simulink model "ModelInterleavedBoostPFCController"  (R2026a)
settings: Solver=ode23t  StopTime=0.02  MaxStep=1e-5  AbsTol=1e-3
PreLoadFcn:
  | InterleavedBoostPFCDefaultInputParameters;
model workspace (MAT data in the model file):
  ConverterKey : string (value not decoded)
undefined symbols (not defined in the file or in its folder): interleavedController, interleavedDesign, Vref
libraries: fl_lib x32, ee_lib x21, nesl_utility x19, ConverterLibrary x1
(part 3 of 3)

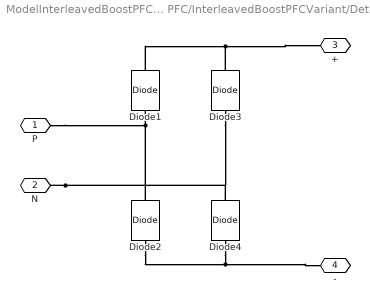
== system ModelInterleavedBoostPFCController/Interleaved Boost PFC/InterleavedBoostPFCVariant/DetailedModel/RectifierBridge/TabulatedDiode ==
  Diode1 : ee_lib/Semiconductors & Converters/Diode  PartSpecification="{\"CollectionId\":\"SimscapeElectrical\",\"CollectionVersion\":\"1.0.0\",\"DatasetId\":\"Infineon|IDW80C65D1|simscape.electrical.diode\",\"DisplayName\":\"Infineon:IDW80C65D1\"}"  ModelType=ee.enum.diode.modelType.tabulated  TableType=ee.enum.diode.tableType.IfMat  IfMat=[0.0001 0.0001 0.1601 0.6065 1.9426 5.4603 12.2546 21.9425 34.4556 49.1982 64.7538 83.3404;0.3114 0.8503 2.3479 5.2232 9.8335 15.9488 23.5801 32.5233 43.1998 54.3228 66.653 79.8979] % Datasheet derived A  VfMat=[.9, 1.15, 1.25, 1.5, 1.75, 2.17, 2.6, 2.85; .58, .68, .75, 1.1, 1.38, 1.77, 2.27, 2.7] % Parameter not set V  TjVec=[25 175] % Datasheet derived degC  VfVec=[0.3258 0.4465 0.5672 0.6878 0.8085 0.9292 1.0498 1.1705 1.2912 1.4118 1.5325 1.6532] % Datasheet derived V  IfVec=[.1, .2, .5, 1, 2, 4, 7, 10] % Parameter not set A  IrMat=[1e-06, 2e-06, 5e-06, 1e-05, 2.5e-05, 5e-05, .0001; 2e-06, 5e-06, 1e-05, 4e-05, 8e-05, .0002, .0005] % Parameter not set A  VrMat=[10, 100, 200, 250, 300, 325, 350; 10, 70, 160, 220, 270, 300, 320] % Parameter not set V  VrVec=[10, 20, 40, 50, 70, 80, 100] % Parameter not set V  IrVec=[1e-06, 2e-06, 5e-06, 1e-05, 2e-05, 5e-05, .0001] % Parameter not set A  Vf=0.6 % Parameter not set V  Ron=0.3 % Parameter not set Ohm  Goff=1e-08 % Parameter not set S  prmExp=ee.enum.diode.expParam.useTwo  I12=[.0137, .545] % Parameter not set A  V12=[.6, .7] % Parameter not set V  RS=0 % Parameter not set Ohm  Tmeas=298.15 % Parameter not set K  IS=1e-12 % Parameter not set A  ec=1 % Parameter not set  I1=0.0137 % Parameter not set A  V1=0.6 % Parameter not set V  N_series=1 % Parameter not set  N_parallel=1 % Parameter not set  ZenerEnable=false % Parameter not set  Rz=0.3 % Parameter not set Ohm  BV=inf % Parameter not set V  C_param=ee.enum.diode.capParam.fixed  CJ=5 pF  CJ0=5 % Parameter not set pF  Vvec=[.1, 10, 100] % Parameter not set V  Cvec=[3.5, 1, .4] % Parameter not set pF  VJ=1 % Parameter not set V  Mgrad=0.5 % Parameter not set  FC=0.5 % Parameter not set  Q_param=ee.enum.diode.recoveryParam.off  iRM=-7.15 % Parameter not set A  iF=4 % Parameter not set A  didt=-750 % Parameter not set A/us  trr_factor=3 % Parameter not set  trr=115 % Parameter not set ns  Qrr=150 % Parameter not set nA*s  Vr=-600 % Parameter not set V  Ls=150 % Parameter not set nH  Erec=0.03 % Parameter not set J  TT=50 % Parameter not set ns  tau=100 % Parameter not set ns  T_param=ee.enum.diode.temperatureParam.off  Tdevice=simTemp_K K  I1_T2=0.245 % Parameter not set A  V1_T2=0.5 % Parameter not set V  IS_T2=1.25e-7 % Parameter not set A  Tmeas2=125 % Parameter not set degC  XTI_param=ee.enum.diode.xtiParam.pn  XTI=3 % Parameter not set  EG_param=ee.enum.diode.egapParam.material_si  EG=1.11 % Parameter not set eV  dBVdT=0 % Parameter not set V/K  enable_fault_input=simscape.enum.onoff.off  i_specify=off  i_priority=None  i=0 A  i_nominal_specify=off  i_nominal_value=1  i_nominal_unit=A  v_specify=off  v_priority=None  v=0 V  v_nominal_specify=off  v_nominal_value=1  v_nominal_unit=V  v_capacitor_specify=off  v_capacitor_priority=None  v_capacitor=0 V  v_capacitor_nominal_specify=off  v_capacitor_nominal_value=1  v_capacitor_nominal_unit=V  Qj_specify=off  Qj_priority=High  Qj=0 C  Qj_nominal_specify=off  Qj_nominal_value=1  Qj_nominal_unit=C  i_diode_specify=off  i_diode_priority=None  i_diode=0 A  i_diode_nominal_specify=off  i_diode_nominal_value=1  i_diode_nominal_unit=A  v_diode_specify=off  v_diode_priority=None  v_diode=0 V  v_diode_nominal_specify=off  v_diode_nominal_value=1  v_diode_nominal_unit=V  i_capacitor_specify=off  i_capacitor_priority=None  i_capacitor=0 A  i_capacitor_nominal_specify=off  i_capacitor_nominal_value=1  i_capacitor_nominal_unit=A  fidelity_level=ee.enum.diode.fidelity.includeChargeDyn  rec_loss_model=ee.enum.diode.reverseRecoveryModel.fixed  ErecVal=0 % Parameter not set J  scaleWithIandV=true % Parameter not set  ErecMat=zeros(2, 3) % Parameter not set J  ErecMat3D=zeros(2, 3, 2) J  TjrecVec=[298.15, 398.15] % Parameter not set K  IfrecVec=[.1, 1, 10] % Parameter not set A  IrecVal=10 % Parameter not set A  VrecVal=10 % Parameter not set V  VrecVec=[0, 100] V  tFilter=1 / 1000 / 100 % Parameter not set s  thermal_network_parameterization=ee.enum.thermalNetworkTopology.junctionCase  Rth=[0, 10] % Parameter not set K/W  Rth_Cauer=[1, 3, 10] % Parameter not set K/W  Rth_Foster=[.08, .14, .22, .16] % Parameter not set K/W  thermal_mass_parameterization=ee.enum.thermalNetwork.timeconstant  thermal_mass=[0, 1] % Parameter not set J/K  thermal_mass_Cauer=[.1, .3, 1] % Parameter not set J/K  thermal_mass_Foster=[.001, .005, .05, .5] % Parameter not set J/K  thermal_time_constant=[0, 10] % Parameter not set s  thermal_time_constant_Cauer=[1, 3, 10] % Parameter not set s  thermal_time_constant_Foster=[7e-05, .0007, .01, .08] % Parameter not set s  thermal_mass_initial_temperatures=[25, 25] % Parameter not set degC  thermal_mass_initial_temperatures_Cauer=[25, 25, 25] % Parameter not set degC  junction_thermal_mass=0.01 % Parameter not set J/K  Tvec_initial_Foster=[25, 25, 25, 25] % Parameter not set degC  no_thermal_network=0 % Parameter not set  junction_temperature_specify=off  junction_temperature_priority=None  junction_temperature=25 degC  junction_temperature_nominal_specify=off  junction_temperature_nominal_value=1  junction_temperature_nominal_unit=degC
      settings: AttributesFormatString=Infineon:IDW80C65D1
  Diode2 : ee_lib/Semiconductors & Converters/Diode  ModelType=ee.enum.diode.modelType.tabulated  TableType=ee.enum.diode.tableType.IfMat  IfMat=[0.0001 0.0001 0.1601 0.6065 1.9426 5.4603 12.2546 21.9425 34.4556 49.1982 64.7538 83.3404;0.3114 0.8503 2.3479 5.2232 9.8335 15.9488 23.5801 32.5233 43.1998 54.3228 66.653 79.8979] % Datasheet derived A  VfMat=[.9, 1.15, 1.25, 1.5, 1.75, 2.17, 2.6, 2.85; .58, .68, .75, 1.1, 1.38, 1.77, 2.27, 2.7] % Parameter not set V  TjVec=[25 175] % Datasheet derived degC  VfVec=[0.3258 0.4465 0.5672 0.6878 0.8085 0.9292 1.0498 1.1705 1.2912 1.4118 1.5325 1.6532] % Datasheet derived V  IfVec=[.1, .2, .5, 1, 2, 4, 7, 10] % Parameter not set A  IrMat=[1e-06, 2e-06, 5e-06, 1e-05, 2.5e-05, 5e-05, .0001; 2e-06, 5e-06, 1e-05, 4e-05, 8e-05, .0002, .0005] % Parameter not set A  VrMat=[10, 100, 200, 250, 300, 325, 350; 10, 70, 160, 220, 270, 300, 320] % Parameter not set V  VrVec=[10, 20, 40, 50, 70, 80, 100] % Parameter not set V  IrVec=[1e-06, 2e-06, 5e-06, 1e-05, 2e-05, 5e-05, .0001] % Parameter not set A  Vf=0.6 % Parameter not set V  Ron=0.3 % Parameter not set Ohm  Goff=1e-08 % Parameter not set S  prmExp=ee.enum.diode.expParam.useTwo  I12=[.0137, .545] % Parameter not set A  V12=[.6, .7] % Parameter not set V  RS=0 % Parameter not set Ohm  Tmeas=298.15 % Parameter not set K  IS=1e-12 % Parameter not set A  ec=1 % Parameter not set  I1=0.0137 % Parameter not set A  V1=0.6 % Parameter not set V  N_series=1 % Parameter not set  N_parallel=1 % Parameter not set  ZenerEnable=false % Parameter not set  Rz=0.3 % Parameter not set Ohm  BV=inf % Parameter not set V  C_param=ee.enum.diode.capParam.fixed  CJ=5 pF  CJ0=5 % Parameter not set pF  Vvec=[.1, 10, 100] % Parameter not set V  Cvec=[3.5, 1, .4] % Parameter not set pF  VJ=1 % Parameter not set V  Mgrad=0.5 % Parameter not set  FC=0.5 % Parameter not set  Q_param=ee.enum.diode.recoveryParam.off  iRM=-7.15 % Parameter not set A  iF=4 % Parameter not set A  didt=-750 % Parameter not set A/us  trr_factor=3 % Parameter not set  trr=115 % Parameter not set ns  Qrr=150 % Parameter not set nA*s  Vr=-600 % Parameter not set V  Ls=150 % Parameter not set nH  Erec=0.03 % Parameter not set J  TT=50 % Parameter not set ns  tau=100 % Parameter not set ns  T_param=ee.enum.diode.temperatureParam.off  Tdevice=simTemp_K K  I1_T2=0.245 % Parameter not set A  V1_T2=0.5 % Parameter not set V  IS_T2=1.25e-7 % Parameter not set A  Tmeas2=125 % Parameter not set degC  XTI_param=ee.enum.diode.xtiParam.pn  XTI=3 % Parameter not set  EG_param=ee.enum.diode.egapParam.material_si  EG=1.11 % Parameter not set eV  dBVdT=0 % Parameter not set V/K  enable_fault_input=simscape.enum.onoff.off  i_specify=off  i_priority=None  i=0 A  i_nominal_specify=off  i_nominal_value=1  i_nominal_unit=A  v_specify=off  v_priority=None  v=0 V  v_nominal_specify=off  v_nominal_value=1  v_nominal_unit=V  v_capacitor_specify=off  v_capacitor_priority=None  v_capacitor=0 V  v_capacitor_nominal_specify=off  v_capacitor_nominal_value=1  v_capacitor_nominal_unit=V  Qj_specify=off  Qj_priority=High  Qj=0 C  Qj_nominal_specify=off  Qj_nominal_value=1  Qj_nominal_unit=C  i_diode_specify=off  i_diode_priority=None  i_diode=0 A  i_diode_nominal_specify=off  i_diode_nominal_value=1  i_diode_nominal_unit=A  v_diode_specify=off  v_diode_priority=None  v_diode=0 V  v_diode_nominal_specify=off  v_diode_nominal_value=1  v_diode_nominal_unit=V  i_capacitor_specify=off  i_capacitor_priority=None  i_capacitor=0 A  i_capacitor_nominal_specify=off  i_capacitor_nominal_value=1  i_capacitor_nominal_unit=A  fidelity_level=ee.enum.diode.fidelity.includeChargeDyn  rec_loss_model=ee.enum.diode.reverseRecoveryModel.fixed  ErecVal=0 % Parameter not set J  scaleWithIandV=true % Parameter not set  ErecMat=zeros(2, 3) % Parameter not set J  ErecMat3D=zeros(2, 3, 2) J  TjrecVec=[298.15, 398.15] % Parameter not set K  IfrecVec=[.1, 1, 10] % Parameter not set A  IrecVal=10 % Parameter not set A  VrecVal=10 % Parameter not set V  VrecVec=[0, 100] V  tFilter=1 / 1000 / 100 % Parameter not set s  thermal_network_parameterization=ee.enum.thermalNetworkTopology.junctionCase  Rth=[0, 10] % Parameter not set K/W  Rth_Cauer=[1, 3, 10] % Parameter not set K/W  Rth_Foster=[.08, .14, .22, .16] % Parameter not set K/W  thermal_mass_parameterization=ee.enum.thermalNetwork.timeconstant  thermal_mass=[0, 1] % Parameter not set J/K  thermal_mass_Cauer=[.1, .3, 1] % Parameter not set J/K  thermal_mass_Foster=[.001, .005, .05, .5] % Parameter not set J/K  thermal_time_constant=[0, 10] % Parameter not set s  thermal_time_constant_Cauer=[1, 3, 10] % Parameter not set s  thermal_time_constant_Foster=[7e-05, .0007, .01, .08] % Parameter not set s  thermal_mass_initial_temperatures=[25, 25] % Parameter not set degC  thermal_mass_initial_temperatures_Cauer=[25, 25, 25] % Parameter not set degC  junction_thermal_mass=0.01 % Parameter not set J/K  Tvec_initial_Foster=[25, 25, 25, 25] % Parameter not set degC  no_thermal_network=0 % Parameter not set  junction_temperature_specify=off  junction_temperature_priority=None  junction_temperature=25 degC  junction_temperature_nominal_specify=off  junction_temperature_nominal_value=1  junction_temperature_nominal_unit=degC
  Diode3 : ee_lib/Semiconductors & Converters/Diode  ModelType=ee.enum.diode.modelType.tabulated  TableType=ee.enum.diode.tableType.IfMat  IfMat=[0.0001 0.0001 0.1601 0.6065 1.9426 5.4603 12.2546 21.9425 34.4556 49.1982 64.7538 83.3404;0.3114 0.8503 2.3479 5.2232 9.8335 15.9488 23.5801 32.5233 43.1998 54.3228 66.653 79.8979] % Datasheet derived A  VfMat=[.9, 1.15, 1.25, 1.5, 1.75, 2.17, 2.6, 2.85; .58, .68, .75, 1.1, 1.38, 1.77, 2.27, 2.7] % Parameter not set V  TjVec=[25 175] % Datasheet derived degC  VfVec=[0.3258 0.4465 0.5672 0.6878 0.8085 0.9292 1.0498 1.1705 1.2912 1.4118 1.5325 1.6532] % Datasheet derived V  IfVec=[.1, .2, .5, 1, 2, 4, 7, 10] % Parameter not set A  IrMat=[1e-06, 2e-06, 5e-06, 1e-05, 2.5e-05, 5e-05, .0001; 2e-06, 5e-06, 1e-05, 4e-05, 8e-05, .0002, .0005] % Parameter not set A  VrMat=[10, 100, 200, 250, 300, 325, 350; 10, 70, 160, 220, 270, 300, 320] % Parameter not set V  VrVec=[10, 20, 40, 50, 70, 80, 100] % Parameter not set V  IrVec=[1e-06, 2e-06, 5e-06, 1e-05, 2e-05, 5e-05, .0001] % Parameter not set A  Vf=0.6 % Parameter not set V  Ron=0.3 % Parameter not set Ohm  Goff=1e-08 % Parameter not set S  prmExp=ee.enum.diode.expParam.useTwo  I12=[.0137, .545] % Parameter not set A  V12=[.6, .7] % Parameter not set V  RS=0 % Parameter not set Ohm  Tmeas=298.15 % Parameter not set K  IS=1e-12 % Parameter not set A  ec=1 % Parameter not set  I1=0.0137 % Parameter not set A  V1=0.6 % Parameter not set V  N_series=1 % Parameter not set  N_parallel=1 % Parameter not set  ZenerEnable=false % Parameter not set  Rz=0.3 % Parameter not set Ohm  BV=inf % Parameter not set V  C_param=ee.enum.diode.capParam.fixed  CJ=5 pF  CJ0=5 % Parameter not set pF  Vvec=[.1, 10, 100] % Parameter not set V  Cvec=[3.5, 1, .4] % Parameter not set pF  VJ=1 % Parameter not set V  Mgrad=0.5 % Parameter not set  FC=0.5 % Parameter not set  Q_param=ee.enum.diode.recoveryParam.off  iRM=-7.15 % Parameter not set A  iF=4 % Parameter not set A  didt=-750 % Parameter not set A/us  trr_factor=3 % Parameter not set  trr=115 % Parameter not set ns  Qrr=150 % Parameter not set nA*s  Vr=-600 % Parameter not set V  Ls=150 % Parameter not set nH  Erec=0.03 % Parameter not set J  TT=50 % Parameter not set ns  tau=100 % Parameter not set ns  T_param=ee.enum.diode.temperatureParam.off  Tdevice=simTemp_K K  I1_T2=0.245 % Parameter not set A  V1_T2=0.5 % Parameter not set V  IS_T2=1.25e-7 % Parameter not set A  Tmeas2=125 % Parameter not set degC  XTI_param=ee.enum.diode.xtiParam.pn  XTI=3 % Parameter not set  EG_param=ee.enum.diode.egapParam.material_si  EG=1.11 % Parameter not set eV  dBVdT=0 % Parameter not set V/K  enable_fault_input=simscape.enum.onoff.off  i_specify=off  i_priority=None  i=0 A  i_nominal_specify=off  i_nominal_value=1  i_nominal_unit=A  v_specify=off  v_priority=None  v=0 V  v_nominal_specify=off  v_nominal_value=1  v_nominal_unit=V  v_capacitor_specify=off  v_capacitor_priority=None  v_capacitor=0 V  v_capacitor_nominal_specify=off  v_capacitor_nominal_value=1  v_capacitor_nominal_unit=V  Qj_specify=off  Qj_priority=High  Qj=0 C  Qj_nominal_specify=off  Qj_nominal_value=1  Qj_nominal_unit=C  i_diode_specify=off  i_diode_priority=None  i_diode=0 A  i_diode_nominal_specify=off  i_diode_nominal_value=1  i_diode_nominal_unit=A  v_diode_specify=off  v_diode_priority=None  v_diode=0 V  v_diode_nominal_specify=off  v_diode_nominal_value=1  v_diode_nominal_unit=V  i_capacitor_specify=off  i_capacitor_priority=None  i_capacitor=0 A  i_capacitor_nominal_specify=off  i_capacitor_nominal_value=1  i_capacitor_nominal_unit=A  fidelity_level=ee.enum.diode.fidelity.includeChargeDyn  rec_loss_model=ee.enum.diode.reverseRecoveryModel.fixed  ErecVal=0 % Parameter not set J  scaleWithIandV=true % Parameter not set  ErecMat=zeros(2, 3) % Parameter not set J  ErecMat3D=zeros(2, 3, 2) J  TjrecVec=[298.15, 398.15] % Parameter not set K  IfrecVec=[.1, 1, 10] % Parameter not set A  IrecVal=10 % Parameter not set A  VrecVal=10 % Parameter not set V  VrecVec=[0, 100] V  tFilter=1 / 1000 / 100 % Parameter not set s  thermal_network_parameterization=ee.enum.thermalNetworkTopology.junctionCase  Rth=[0, 10] % Parameter not set K/W  Rth_Cauer=[1, 3, 10] % Parameter not set K/W  Rth_Foster=[.08, .14, .22, .16] % Parameter not set K/W  thermal_mass_parameterization=ee.enum.thermalNetwork.timeconstant  thermal_mass=[0, 1] % Parameter not set J/K  thermal_mass_Cauer=[.1, .3, 1] % Parameter not set J/K  thermal_mass_Foster=[.001, .005, .05, .5] % Parameter not set J/K  thermal_time_constant=[0, 10] % Parameter not set s  thermal_time_constant_Cauer=[1, 3, 10] % Parameter not set s  thermal_time_constant_Foster=[7e-05, .0007, .01, .08] % Parameter not set s  thermal_mass_initial_temperatures=[25, 25] % Parameter not set degC  thermal_mass_initial_temperatures_Cauer=[25, 25, 25] % Parameter not set degC  junction_thermal_mass=0.01 % Parameter not set J/K  Tvec_initial_Foster=[25, 25, 25, 25] % Parameter not set degC  no_thermal_network=0 % Parameter not set  junction_temperature_specify=off  junction_temperature_priority=None  junction_temperature=25 degC  junction_temperature_nominal_specify=off  junction_temperature_nominal_value=1  junction_temperature_nominal_unit=degC
  Diode4 : ee_lib/Semiconductors & Converters/Diode  ModelType=ee.enum.diode.modelType.tabulated  TableType=ee.enum.diode.tableType.IfMat  IfMat=[0.0001 0.0001 0.1601 0.6065 1.9426 5.4603 12.2546 21.9425 34.4556 49.1982 64.7538 83.3404;0.3114 0.8503 2.3479 5.2232 9.8335 15.9488 23.5801 32.5233 43.1998 54.3228 66.653 79.8979] % Datasheet derived A  VfMat=[.9, 1.15, 1.25, 1.5, 1.75, 2.17, 2.6, 2.85; .58, .68, .75, 1.1, 1.38, 1.77, 2.27, 2.7] % Parameter not set V  TjVec=[25 175] % Datasheet derived degC  VfVec=[0.3258 0.4465 0.5672 0.6878 0.8085 0.9292 1.0498 1.1705 1.2912 1.4118 1.5325 1.6532] % Datasheet derived V  IfVec=[.1, .2, .5, 1, 2, 4, 7, 10] % Parameter not set A  IrMat=[1e-06, 2e-06, 5e-06, 1e-05, 2.5e-05, 5e-05, .0001; 2e-06, 5e-06, 1e-05, 4e-05, 8e-05, .0002, .0005] % Parameter not set A  VrMat=[10, 100, 200, 250, 300, 325, 350; 10, 70, 160, 220, 270, 300, 320] % Parameter not set V  VrVec=[10, 20, 40, 50, 70, 80, 100] % Parameter not set V  IrVec=[1e-06, 2e-06, 5e-06, 1e-05, 2e-05, 5e-05, .0001] % Parameter not set A  Vf=0.6 % Parameter not set V  Ron=0.3 % Parameter not set Ohm  Goff=1e-08 % Parameter not set S  prmExp=ee.enum.diode.expParam.useTwo  I12=[.0137, .545] % Parameter not set A  V12=[.6, .7] % Parameter not set V  RS=0 % Parameter not set Ohm  Tmeas=298.15 % Parameter not set K  IS=1e-12 % Parameter not set A  ec=1 % Parameter not set  I1=0.0137 % Parameter not set A  V1=0.6 % Parameter not set V  N_series=1 % Parameter not set  N_parallel=1 % Parameter not set  ZenerEnable=false % Parameter not set  Rz=0.3 % Parameter not set Ohm  BV=inf % Parameter not set V  C_param=ee.enum.diode.capParam.fixed  CJ=5 pF  CJ0=5 % Parameter not set pF  Vvec=[.1, 10, 100] % Parameter not set V  Cvec=[3.5, 1, .4] % Parameter not set pF  VJ=1 % Parameter not set V  Mgrad=0.5 % Parameter not set  FC=0.5 % Parameter not set  Q_param=ee.enum.diode.recoveryParam.off  iRM=-7.15 % Parameter not set A  iF=4 % Parameter not set A  didt=-750 % Parameter not set A/us  trr_factor=3 % Parameter not set  trr=115 % Parameter not set ns  Qrr=150 % Parameter not set nA*s  Vr=-600 % Parameter not set V  Ls=150 % Parameter not set nH  Erec=0.03 % Parameter not set J  TT=50 % Parameter not set ns  tau=100 % Parameter not set ns  T_param=ee.enum.diode.temperatureParam.off  Tdevice=simTemp_K K  I1_T2=0.245 % Parameter not set A  V1_T2=0.5 % Parameter not set V  IS_T2=1.25e-7 % Parameter not set A  Tmeas2=125 % Parameter not set degC  XTI_param=ee.enum.diode.xtiParam.pn  XTI=3 % Parameter not set  EG_param=ee.enum.diode.egapParam.material_si  EG=1.11 % Parameter not set eV  dBVdT=0 % Parameter not set V/K  enable_fault_input=simscape.enum.onoff.off  i_specify=off  i_priority=None  i=0 A  i_nominal_specify=off  i_nominal_value=1  i_nominal_unit=A  v_specify=off  v_priority=None  v=0 V  v_nominal_specify=off  v_nominal_value=1  v_nominal_unit=V  v_capacitor_specify=off  v_capacitor_priority=None  v_capacitor=0 V  v_capacitor_nominal_specify=off  v_capacitor_nominal_value=1  v_capacitor_nominal_unit=V  Qj_specify=off  Qj_priority=High  Qj=0 C  Qj_nominal_specify=off  Qj_nominal_value=1  Qj_nominal_unit=C  i_diode_specify=off  i_diode_priority=None  i_diode=0 A  i_diode_nominal_specify=off  i_diode_nominal_value=1  i_diode_nominal_unit=A  v_diode_specify=off  v_diode_priority=None  v_diode=0 V  v_diode_nominal_specify=off  v_diode_nominal_value=1  v_diode_nominal_unit=V  i_capacitor_specify=off  i_capacitor_priority=None  i_capacitor=0 A  i_capacitor_nominal_specify=off  i_capacitor_nominal_value=1  i_capacitor_nominal_unit=A  fidelity_level=ee.enum.diode.fidelity.includeChargeDyn  rec_loss_model=ee.enum.diode.reverseRecoveryModel.fixed  ErecVal=0 % Parameter not set J  scaleWithIandV=true % Parameter not set  ErecMat=zeros(2, 3) % Parameter not set J  ErecMat3D=zeros(2, 3, 2) J  TjrecVec=[298.15, 398.15] % Parameter not set K  IfrecVec=[.1, 1, 10] % Parameter not set A  IrecVal=10 % Parameter not set A  VrecVal=10 % Parameter not set V  VrecVec=[0, 100] V  tFilter=1 / 1000 / 100 % Parameter not set s  thermal_network_parameterization=ee.enum.thermalNetworkTopology.junctionCase  Rth=[0, 10] % Parameter not set K/W  Rth_Cauer=[1, 3, 10] % Parameter not set K/W  Rth_Foster=[.08, .14, .22, .16] % Parameter not set K/W  thermal_mass_parameterization=ee.enum.thermalNetwork.timeconstant  thermal_mass=[0, 1] % Parameter not set J/K  thermal_mass_Cauer=[.1, .3, 1] % Parameter not set J/K  thermal_mass_Foster=[.001, .005, .05, .5] % Parameter not set J/K  thermal_time_constant=[0, 10] % Parameter not set s  thermal_time_constant_Cauer=[1, 3, 10] % Parameter not set s  thermal_time_constant_Foster=[7e-05, .0007, .01, .08] % Parameter not set s  thermal_mass_initial_temperatures=[25, 25] % Parameter not set degC  thermal_mass_initial_temperatures_Cauer=[25, 25, 25] % Parameter not set degC  junction_thermal_mass=0.01 % Parameter not set J/K  Tvec_initial_Foster=[25, 25, 25, 25] % Parameter not set degC  no_thermal_network=0 % Parameter not set  junction_temperature_specify=off  junction_temperature_priority=None  junction_temperature=25 degC  junction_temperature_nominal_specify=off  junction_temperature_nominal_value=1  junction_temperature_nominal_unit=degC
  P : PMIOPort  Side=Left
  N : PMIOPort  Port=2  Side=Left
  + : PMIOPort  Port=3  Side=Right
  - : PMIOPort  Port=4  Side=Right
  connections:
  Diode1/LConn1 -- P/RConn1 -- Diode2/RConn1
  N/RConn1 -- Diode4/RConn1 -- Diode3/LConn1
  Diode4/LConn1 -- -/RConn1 -- Diode2/LConn1
  Diode3/RConn1 -- +/RConn1 -- Diode1/RConn1
